simulink model "TB04_StageB_ClosedLoop"  (R2025a)
settings: Solver=FixedStepDiscrete  StartTime=0  StopTime=TB.t_end  FixedStep=TB.dt  RelTol=1e-3
InitFcn:
  | % 모델과 같은 폴더의 초기화 스크립트를 실행해 P(설계 파라미터)와 TB(시험 조건)를 만든다.
  | run(fullfile(fileparts(get_param(bdroot, 'FileName')), 'TB04_init.m'));
values from neighbouring files (symbols this model uses):
  TB = struct()    [TB04_init.m]
libraries: fl_lib x56, nesl_utility x23
(part 2 of 2)

== system TB04_StageB_ClosedLoop/StageB_Regulator/HBridge/QB_low ==
  note: 스위치 셀: 이상 스위치(R_on, G_off) + 역병렬 바디 다이오드(Vf, R_d) + 출력용량 C_oss
      | 게이트: 전역 태그 "gB_BL" (> 0.5 이면 도통)
  C_oss : fl_lib/Electrical/Electrical Elements/Capacitor  c=Coss F  r=1e-6 Ohm  g=0 1/Ohm  i_specify=off  i_priority=None  i=0 A  i_nominal_specify=off  i_nominal_value=1  i_nominal_unit=A  v_specify=off  v_priority=None  v=0 V  v_nominal_specify=off  v_nominal_value=1  v_nominal_unit=V  vc_specify=off  vc_priority=High  vc=0 V  vc_nominal_specify=off  vc_nominal_value=1  vc_nominal_unit=V
  D_body : fl_lib/Electrical/Electrical Elements/Diode  Vf=Vf V  Ron=Rd Ohm  Goff=Goffd 1/Ohm  i_specify=off  i_priority=None  i=0 A  i_nominal_specify=off  i_nominal_value=1  i_nominal_unit=A  v_specify=off  v_priority=None  v=0 V  v_nominal_specify=off  v_nominal_value=1  v_nominal_unit=V
  Gate_PS : nesl_utility/Simulink-PS Converter  PhysicalDomain=network_engine_domain  SubClassName=ps_input  LeftPortType=input  RightPortType=output  PseudoPeriodic=off  Frequencies=[]  NoiseDistribution=none  NoiseParameters=[]  Unit=1  AffineConversion=off  FilteringAndDerivatives=zero  SimscapeFilterOrder=1  InputFilterTimeConstant=0.001  UdotUserProvided=0
  SW : fl_lib/Electrical/Electrical Elements/Switch  R_closed=Ron Ohm  G_open=Goff 1/Ohm  Threshold=0.5  i_specify=off  i_priority=None  i=0 A  i_nominal_specify=off  i_nominal_value=1  i_nominal_unit=A  v_specify=off  v_priority=None  v=0 V  v_nominal_specify=off  v_nominal_value=1  v_nominal_unit=V
  D : PMIOPort  Side=Left
  S : PMIOPort  Port=2  Side=Right
  wires:
  [gB_BL] -> Gate_PS/1
  connections:
  Gate_PS/RConn1 -- SW/RConn1
  SW/LConn1 -- D/RConn1 -- D_body/RConn1 -- C_oss/LConn1
  SW/RConn2 -- D_body/LConn1 -- S/RConn1 -- C_oss/RConn1

== matlab function TB04_StageB_ClosedLoop/Controller_StageB/Adopted_Controller ==
  data: t input; u output; y input; prm input; init input; tab input; smp input; dg output
function [u, dg] = prism_ctrl_sampler(t, y, prm, init, tab, smp)
%#codegen
%PRISM_CTRL_SAMPLER  채택 제어기의 표본화 실행기(MATLAB Function 블록의 진입 함수).
%
%   모델 전체를 적분 간격 dt 하나로 돌리고(다중 속도 없음), 이 함수가 반송파 최댓값 시점
%   (k = round(t/dt)가 Np의 배수, 5 µs마다)에만 제어기를 한 번 계산한다. 그 밖의 간격에서는 직전 출력을 유지한다.
%   계산 결과는 모델의 Delay 블록(Np 간격 = 5 µs)을 거쳐 게이트 생성기에 들어가므로, 검증 모델과 같이
%   표본 → 계산 → 5 µs 뒤 적용 순서가 된다.
%
%   입력  t     시각 [s] (Digital Clock)
%         y     [i_p v_s v_bus i_h v_link V_bat i_link_avg φ_c0 φ_c1]  (prism_stageB_controller 설명 참고)
%         prm, init, tab  제어기 상수(prism_hub_params: P.ctrl_prm, 초기상태, 데드타임 교정표)
%         smp   [dt Np]
%   출력  u     [PWM 비교값; DAB 유효 위상]   dg  [m 지령; 링크전류 지령; 브리지 전류지령; ρ̂; ε̂; 예측 링크전류]

persistent uh dgh
if isempty(uh)
    uh = [init(3); 0];
    dgh = zeros(6, 1);
end
k = round(t/smp(1));
if mod(k, round(smp(2))) == 0
    [uh, dgh] = prism_stageB_controller(y, prm, init, tab);
end
u = uh;
dg = dgh;
end

function [u, dg] = prism_stageB_controller(y, prm, init, tab)
%#codegen
%PRISM_STAGEB_CONTROLLER  Stage B 채택 제어기 1회 계산(제어주기 5 µs, 반송파 최댓값에서 표본).
%
%  검증 코드(model_stage_b_switching.run_core의 제어 부분)와 같은 법칙이다.
%   (1) 1주기 예측: 고속 상태 [i_p, v_s, i_h]를 직전 변조율로 5 µs 앞까지 공칭 모델로 적분(중점법 5단계)
%   (2) 상태궤환 + 버스전압 적분 → 브리지 전류지령(±84 A 포화, 역포화 보정)
%   (3) 내부 전류 법칙 → 변조율 m(±0.95)
%   (4) 링크전압 PI + 소비전류 앞먹임 → DAB 링크전류 지령(정격 80 A·8 kW·SPS 한계)
%   (5) DAB 링크전류 → 위상: 누설 인덕턴스 −10 % 기준 앞먹임 + 측정 전류비 ρ̂ 보정 + 저전류 가산 보정 ε̂
%   (6) H-브리지 데드타임 보상: 교정표 × 전류 스케줄 κ(20 A 이하 0.6 → 80 A 1.0)
%
%  입력
%   y    = [i_p v_s v_bus i_h v_link V_bat i_link_avg ph_c0 ph_c1]  (표본값)
%          i_link_avg : 직전 제어주기의 DAB 링크 직류전류 평균(측정)
%          ph_c0/ph_c1: 그 주기의 두 반주기 중심에서 적용된 유효 위상(게이트 생성기가 기록)
%   prm  = 상수 벡터(prism_hub_params의 P.ctrl_prm)
%           1 L  2 Cs  3 Cb  4 R  5 Lh  6 Rh  7 Clink  8 Ts  9 vref  10 vlink  11 mmax  12 refmax
%          13 link_max  14 power_max  15 link_bw  16 inner_tau  17 Ldab  18 fs  19 turns  20 phmax
%          21–25 K  26 lmin(0.9)  27 ρ̂ 이득  28 ρ̂ 최소 전류  29 ε̂ 이득  30 ε̂ 상한
%          31 κ 경부하 비율  32 κ 시작 전류  33 κ 1 도달 전류  34 교정표 기준 링크전압  35 예측 단계 수
%          36 예측 사용(1)  37 데드타임 보상 사용(1)
%   init = [q0 q_link0 m0 i_link0]   (평형점에서 시작: 적분기가 지령 = i_p가 되도록)
%   tab  = [i_grid; E(i)]            데드타임 교정표(전류별 상승 전이 한 번의 전압·시간 손실)
%  출력
%   u  = [PWM 비교값(데드타임 보상 후); DAB 유효 위상 지령 rad]
%   dg = [m 지령(보상 전); 링크전류 지령; 브리지 전류지령; ρ̂; ε̂; 예측 링크전류]

persistent q qlink mprev rho epsA vbprev started
if isempty(started)
    q = init(1); qlink = init(2); mprev = init(3); rho = 1; epsA = 0; vbprev = y(3); started = 1;
end

L = prm(1); Cs = prm(2); R = prm(4); Lh = prm(5); Rh = prm(6); Clink = prm(7); Ts = prm(8);
vref = prm(9); vlink = prm(10); mmax = prm(11); refmax = prm(12);
link_max = prm(13); power_max = prm(14); link_bw = prm(15); itau = prm(16);
Ldab = prm(17); fs = prm(18); turns = prm(19); phmax = prm(20);
K = prm(21:25);
lmin = prm(26); est_g = prm(27); est_min = prm(28); eps_g = prm(29); eps_max = prm(30);
k_scale = prm(31); k_from = prm(32); k_full = prm(33); Vtab = prm(34); nsub = prm(35);

ip = y(1); vs = y(2); vb = y(3); ih = y(4); vl = y(5); vbat = y(6);
il_meas = y(7); ph_c0 = y(8); ph_c1 = y(9);

% ---- (1) 1주기 예측 -----------------------------------------------------------------
sip = ip; svs = vs; sih = ih;
if prm(36) > 0.5
    m = mprev; h = Ts/nsub;
    for s = 1:nsub
        a1 = (vbat/2 - R*sip + svs - vb)/L;
        a2 = (sih - sip)/Cs;
        a3 = (m*vl - svs - Rh*sih)/Lh;
        mp = sip + 0.5*h*a1;  mv = svs + 0.5*h*a2;  mh = sih + 0.5*h*a3;
        b1 = (vbat/2 - R*mp + mv - vb)/L;
        b2 = (mh - mp)/Cs;
        b3 = (m*vl - mv - Rh*mh)/Lh;
        sip = sip + h*b1;  svs = svs + h*b2;  sih = sih + h*b3;
    end
end
% ---- (2) 상태궤환 + 적분 -----------------------------------------------------------
raw  = -(K(1)*sip + K(2)*svs + K(3)*vb + K(4)*sih) - K(5)*q;
iref = min(refmax, max(-refmax, raw));
q = q + Ts*(vref - vb) + 0.1*(iref - raw)/(-K(5));
% ---- (3) 내부 전류 법칙 → 변조율 ---------------------------------------------------
vlx = max(vl, 1);                                % (보상 계산용 하한)
mraw = (svs + Rh*sih + Lh/itau*(iref - sih))/vl;
mcmd = min(mmax, max(-mmax, mraw));
% ---- (4) 링크전압 PI + 앞먹임 → DAB 링크전류 지령 ---------------------------------
w = 2*pi*link_bw;
rawlink = mcmd*sih + Clink*(2*0.7*w*(vlink - vl) + w*w*qlink);
sps = max(vb, 0)*turns*phmax*(1 - phmax/pi)/(2*pi*fs*Ldab);
lim = min(min(link_max, sps), power_max/max(vl, 1e-9));
icmd = min(lim, max(-lim, rawlink));
qlink = qlink + Ts*(vlink - vl) + 0.1*(icmd - rawlink)/(Clink*w*w);
mprev = mcmd;
% ---- (5) DAB 전류비·저전류 보정 → 위상 ----------------------------------------------
% 직전 주기 두 반주기 중심에 적용된 위상의 예측 전류. 그 위상을 적용할 때 쓰인 버스전압은 직전 표본값이다
% (검증 모델: 반주기 중심에서 그때의 측정 버스전압으로 예측 전류를 계산).
il_pred = 0.5*(ipred(ph_c0, vbprev, turns, fs, Ldab, lmin) + ipred(ph_c1, vbprev, turns, fs, Ldab, lmin));
vbprev = vb;
dph = abs(ph_c1 - ph_c0);
if abs(il_pred) >= est_min && il_meas*il_pred > 0 && dph < 0.035
    rho = rho + est_g*(il_meas/il_pred - rho);
    rho = min(max(rho, 0.75), 1.25);
end
if eps_g > 0
    if abs(il_pred) < est_min && dph < 0.035
        epsA = epsA + eps_g*((il_meas - rho*il_pred) - epsA);
    elseif abs(il_pred) >= est_min
        epsA = epsA - eps_g*epsA;
    end
    epsA = min(max(epsA, -eps_max), eps_max);
end
ph_new = phase_ff((icmd - epsA)/rho, vb, turns, fs, Ldab, lmin, phmax);
% ---- (6) H-브리지 데드타임 보상 ----------------------------------------------------
m_pwm = mcmd;
if prm(37) > 0.5
    kap = k_scale + (1 - k_scale)*min(max((abs(sih) - k_from)/max(k_full - k_from, 1e-9), 0), 1);
    m_pwm = mcmd - kap*dt_error_tab(mcmd, sih, vlx, Lh, fs, tab, Vtab)/vlx;
end
u  = [m_pwm; ph_new];
dg = [mcmd; icmd; iref; rho; epsA; il_pred];
end

% ======================================================================================
function i = ipred(ph, vb, turns, fs, Ldab, lb)
% 위상 ph에서 SPS 식이 주는 링크전류(누설 인덕턴스 = 공칭의 lb배 가정)
k = turns*max(vb, 1)/(2*pi*fs*Ldab*lb);
i = k*ph*(1 - abs(ph)/pi);
end

function ph = phase_ff(il, vb, turns, fs, Ldab, lb, phmax)
% 링크전류 → SPS 위상 앞먹임(|φ| ≤ φ_max)
k = turns*max(vb, 1)/(2*pi*fs*Ldab*lb);
a = min(abs(il)/(pi*k/4), 1);
ph = min(pi/2*(1 - sqrt(1 - a)), phmax);
if il < 0, ph = -ph; end
end

function d = dt_error_tab(m, i, V, Lh, f, tab, Vtab)
% 유니폴라 PWM 한 주기의 브리지 평균 전압오차 [V]: 리플 극값 전류에서의 전이별 손실을 교정표에서 읽는다.
sg = 1;
if m < 0, m = -m; i = -i; sg = -1; end
r = V*m*(1 - m)/(4*Lh*f);
imin = i - r; imax = i + r;
d = sg*2*(tab_interp(-imax, tab) - tab_interp(imin, tab))*(V/Vtab)*f;
end

function e = tab_interp(x, tab)
% 선형 보간(범위 밖은 끝값) — numpy.interp와 같음
n = size(tab, 2);
if x <= tab(1, 1), e = tab(2, 1); return; end
if x >= tab(1, n), e = tab(2, n); return; end
lo = 1; hi = n;
while hi - lo > 1
    mid = floor((lo + hi)/2);
    if tab(1, mid) <= x, lo = mid; else, hi = mid; end
end
w = (x - tab(1, lo))/(tab(1, hi) - tab(1, lo));
e = tab(2, lo) + w*(tab(2, hi) - tab(2, lo));
end

== matlab function TB04_StageB_ClosedLoop/DAB_Loss_Model/DAB_Loss ==
  data: t input; iloss output; vl input; il input; iL input; vb input; prm input; ploss0 input
function iloss = prism_dab_loss(t, vl, il, iL, vb, prm, ploss0)
%#codegen
%PRISM_DAB_LOSS  DAB 손실 등가 전류(검증 모델과 같은 손실 모델).
%
%   스위칭 회로의 DAB에는 권선저항 R_dab만 있고 스위칭·자기 손실이 없다. 검증 모델(E12)은 평균모델과 같은
%   방향별 효율 η = 0.96을 쓰기 위해, 직전 제어주기의 평균 링크전력 p̄로 정한 손실
%       P_loss = (1/η − 1)·max(p̄, 0) + (1 − η)·max(−p̄, 0) − R_dab·mean(i_L²)   (0 이상)
%   을 버스에서 끄는 전류 P_loss/v_bus로 넣는다. 이 블록은 같은 계산을 해서 버스의 제어 전류원에 준다.
%   이렇게 하면 정상상태의 DAB 총손실이 검증 모델과 같아, 두 모델의 차이는 스위칭 동작에서만 나온다.
%
%   입력  t 시각, vl 링크전압, il 링크 직류전류(2차 브리지 → 링크), iL 누설 전류, vb 버스전압
%         prm [dt Np η R_dab]   ploss0 초기 손실 [W](평형점 링크전력 기준)
%   출력  iloss  버스에서 끄는 손실 전류 [A]

persistent accP accI2 ploss started
if isempty(started)
    started = 1; accP = 0; accI2 = 0; ploss = ploss0;
end
dt = prm(1); Np = round(prm(2)); eta = prm(3); Rd = prm(4);
k = round(t/dt);
accP = accP + vl*il;
accI2 = accI2 + iL*iL;
if mod(k, Np) == Np - 1                       % 주기 마지막 간격에서 갱신(다음 주기에 적용)
    pbar = accP/Np;
    lossEta = (1/eta - 1)*max(pbar, 0) + (1 - eta)*max(-pbar, 0);
    ploss = max(lossEta - Rd*accI2/Np, 0);
    accP = 0; accI2 = 0;
end
iloss = ploss/max(vb, 1);
end

== matlab function TB04_StageB_ClosedLoop/Gate_StageB/StageB_Gate ==
  data: t input; g output; uc input; ilink input; prm input; init input; aux output
function [g, aux] = prism_gate_stageB(t, uc, ilink, prm, init)
%#codegen
%PRISM_GATE_STAGEB  Stage B 게이트 생성기(적분 간격 dt = 5 ns마다 실행).
%
%  H-브리지 : 유니폴라 PWM. 삼각 반송파 c(t)는 제어주기 시작(표본 시점)에서 +1, 반주기에서 −1.
%             레그 A 상측 목표 = (m > c), 레그 B 상측 목표 = (−m > c). 목표가 바뀌면 두 소자를 데드타임 동안
%             끄고(출력용량 충방전·다이오드 도통은 회로가 정함) 새 소자를 켠다.
%  DAB      : 50 % 구형파 두 풀브리지, 단일 위상천이. 에지는 반송파 반주기 중심 c_j에 대칭(1차 c_j − δ/2,
%             2차 c_j + δ/2, δ = φ·T/2π)으로 놓고, 지령은 도착 후 첫 반주기 중심에서 반영한다.
%             전이 반주기의 위상차를 이전·새 위상의 평균으로 두는 갱신(A ← −A + 2Δ, Δ = (A + δ_new)/2)으로
%             위상이 바뀔 때 변압기 직류 편류가 생기지 않게 한다(검증 코드와 같은 알고리즘).
%             에지 시각은 dt 격자에 반올림하고, 실제 실행 시각으로 다음 반주기의 A를 계산한다.
%  링크전류 : DAB 2차 브리지가 링크로 보내는 직류전류를 제어주기마다 평균해 다음 표본에 넘긴다.
%
%  입력  t      시뮬레이션 시각(Digital Clock, dt 간격)
%        uc     [PWM 비교값; DAB 유효 위상 rad]  (제어기 출력, 전달지연 뒤)
%        ilink  DAB 2차 브리지 → 링크 직류전류 [A](순시)
%        prm    [dt Np td_h(간격 수) td_d(간격 수) T]
%        init   [PWM 비교값 초기값, 위상 초기값, 링크전류 초기값]
%  출력  g      [A상측 A하측 B상측 B하측 | P1 P2 P3 P4 | S1 S2 S3 S4]  (1 = 켬)
%               DAB 브리지: 상태 +1 → 1·4번 켬, −1 → 2·3번 켬(1·2번이 레그 1, 3·4번이 레그 2, 홀수 = 상측)
%        aux    [링크전류 주기 평균; 그 주기 두 반주기 중심의 위상 φ_c0, φ_c1; 반송파; 1차 상태; 2차 상태]

persistent started kA kB tgtA tgtB A ph_tgt p_t s_t p_h s_h p_j s_j p_state s_state p_te s_te ...
           acc il_avg phc0 phc1 lat0 lat1
dt = prm(1); Np = prm(2); ndh = prm(3); ndd = prm(4); T = prm(5);
Nh = round(Np/2);
k  = round(t/dt);                     % 적분 간격 번호(0부터)
t0 = k*dt;

if isempty(started)
    started = 1;
    m0 = init(1); ph0 = init(2);
    c0 = 1;                            % k = 0의 반송파
    tgtA = double(m0 > c0); tgtB = double(-m0 > c0);
    kA = -1e9; kB = -1e9;              % 데드타임 없이 시작
    ph_tgt = ph0;
    d0 = ph0/(2*pi)*T;
    A = d0;
    p_t = [1e30 1e30]; s_t = [1e30 1e30]; p_h = [0 0]; s_h = [0 0];
    p_te = -1; s_te = -1;
    if d0 > 0
        p_j = 1; p_h(1) = -d0/2; p_state = 1;  s_j = 0; s_state = -1;
    elseif d0 < 0
        s_j = 1; s_h(1) = d0/2;  s_state = 1;  p_j = 0; p_state = -1;
    else
        p_j = 0; s_j = 0; p_state = -1; s_state = -1;
    end
    acc = 0; il_avg = init(3); phc0 = ph0; phc1 = ph0; lat0 = ph0; lat1 = ph0;
end

m = uc(1);
ph_tgt = uc(2);

% ---------------- H-브리지 유니폴라 PWM -------------------------------------------------
kin = mod(k, Np);
c = 4*abs(kin/Np - 0.5) - 1;
nA = double(m > c); nB = double(-m > c);
if nA ~= tgtA, tgtA = nA; kA = k; end
if nB ~= tgtB, tgtB = nB; kB = k; end
okA = (k - kA) >= ndh; okB = (k - kB) >= ndh;
gA_hi = double(okA && tgtA == 1); gA_lo = double(okA && tgtA == 0);
gB_hi = double(okB && tgtB == 1); gB_lo = double(okB && tgtB == 0);

% ---------------- DAB 위상 갱신(반주기 중심) --------------------------------------------
if mod(k, Nh) == 0
    j = k/Nh; cj = t0;
    if j >= 1
        jm = mod(j - 1, 2) + 1;
        A = -A + 2*(s_h(jm) - p_h(jm));
    end
    dtg = ph_tgt/(2*pi)*T;
    D = 0.5*(A + dtg);
    jj = mod(j, 2) + 1;
    p_done = p_j > j; s_done = s_j > j;
    if p_done && ~s_done
        s_t(jj) = max(cj, p_h(jj) + D);
    elseif s_done && ~p_done
        p_t(jj) = max(cj, s_h(jj) - D);
    elseif ~p_done && ~s_done
        if D >= 0
            p_t(jj) = cj; s_t(jj) = cj + D;
        else
            s_t(jj) = cj; p_t(jj) = cj - D;
        end
    end
    if p_done, tpj = p_h(jj); else, tpj = p_t(jj); end
    if s_done, tsj = s_h(jj); else, tsj = s_t(jj); end
    D1 = 0.5*(-A + 2*(tsj - tpj) + dtg);
    cn = (j + 1)*Nh*dt;
    p_t(3 - jj) = cn - D1/2; s_t(3 - jj) = cn + D1/2;
    if mod(j, 2) == 0, phc0 = ph_tgt; else, phc1 = ph_tgt; end
end
% ---------------- DAB 에지 실행(가장 가까운 간격에 반올림) ------------------------------
sp = mod(p_j, 2) + 1;
if p_t(sp) < t0 + 0.5*dt
    if mod(p_j, 2) == 0, p_state = 1; else, p_state = -1; end
    p_te = t0; p_h(sp) = t0; p_t(sp) = 1e30; p_j = p_j + 1;
end
ss = mod(s_j, 2) + 1;
if s_t(ss) < t0 + 0.5*dt
    if mod(s_j, 2) == 0, s_state = 1; else, s_state = -1; end
    s_te = t0; s_h(ss) = t0; s_t(ss) = 1e30; s_j = s_j + 1;
end
p_ok = (t0 - p_te) >= ndd*dt - 0.5*dt;
s_ok = (t0 - s_te) >= ndd*dt - 0.5*dt;
gP = [0 0 0 0]; gS = [0 0 0 0];
if p_ok
    if p_state > 0, gP = [1 0 0 1]; else, gP = [0 1 1 0]; end
end
if s_ok
    if s_state > 0, gS = [1 0 0 1]; else, gS = [0 1 1 0]; end
end

% ---------------- 링크전류 주기 평균(표본 직전 간격에서 확정) -------------------------
acc = acc + ilink;
if kin == Np - 1
    il_avg = acc/Np; acc = 0;
    lat0 = phc0; lat1 = phc1;
end

g = [gA_hi gA_lo gB_hi gB_lo gP gS]';
aux = [il_avg; lat0; lat1; c; p_state; s_state];
end
